simulink model "sinePWM"  (R2024b)
settings: Solver=VariableStepAuto  StartTime=0.0  StopTime=0.5  RelTol=1e-3
libraries: spsMosfetLib x4, spsDCVoltageSourceLib x1, spsSeriesRLCBranchLib x1, spsTriangleGeneratorLib x1, spsVoltageMeasurementLib x1, sps_lib x1
settings Model: Creator=lenovo  LastModifiedBy=lenovo

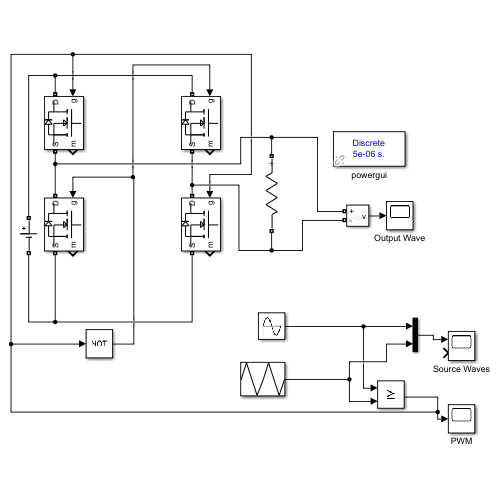
[thumbnail: Simulink's stored preview of the top-level diagram]
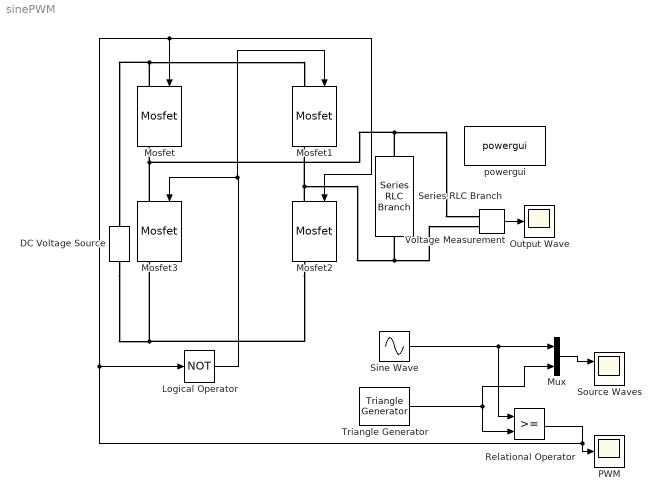
== system sinePWM ==
  DC Voltage Source : spsDCVoltageSourceLib/DC Voltage Source  Amplitude=100  Measurements=None
  Logical Operator : Logic  Operator=NOT  AllPortsSameDT=off  OutDataTypeStr=boolean
  Mosfet{,1..3} (4 alike) : spsMosfetLib/Mosfet  Ron=0.1  Lon=0  Rd=0.01  Vfd=0  IC=0  Rs=1e5  Cs=inf  Measurements=on
  Mux : Mux  Inputs=2
  Output Wave : Scope
  PWM : Scope
  Relational Operator : RelationalOperator  OutDataTypeStr=boolean  RndMeth=Simplest  InputSameDT=off
  Series RLC Branch : spsSeriesRLCBranchLib/Series RLC Branch  LConnTagsString=__new0  RConnTagsString=__new0  BranchType=R  Resistance=1  Inductance=1e-3  SetiL0=off  InitialCurrent=0  Capacitance=1e-6  Setx0=off  InitialVoltage=0  Measurements=None
  Sine Wave : Sin  Frequency=100  SampleTime=0
  Source Waves : Scope  NumInputPorts=2
  Triangle Generator : spsTriangleGeneratorLib/Triangle Generator  Freq=1e1  Phase=90  Ts=0
  Voltage Measurement : spsVoltageMeasurementLib/Voltage Measurement  PhasorSimulation=off  OutputType=Complex  PSBequivalent=0
  powergui : sps_lib/powergui  Priority=1  SimulationMode=Discrete  SampleTime=5e-6  frequency=60  Iterations=50  frequencyindice=0  Pbase=100e6  ErrMax=1e-4  UnitsV=kV  UnitsW=MW  buscounter=0  FunctionMessages=off  echomessages=off  EnableUseOfTLC=off  CurrentSourceSwitches=off  DisableSnubberDevices=off  DisableRonSwitches=off  DisableVfSwitches=off  DisplayEquations=off  AutomaticDiscreteSolvers=off  SolverType=Tustin/Backward Euler (TBE)  Interpol=off  ExternalGateDelay=off  methode=off  Ts=100  x0status=blocks  SPID=on  SwTol=0  HookPort=off  NonlinearTolerance=1e-4  nMaxIteration=100  ContinueOnMaxIteration=off  RestoreLinks=warning  ResistiveCurrentMeasurement=off  Frange=[0:2:500]  Ylog=off  Xlog=on  ShowGrid=off  save=off  variable=ZData  structure=0  ZoomFFT=off  StartTime=0.0  cycles=1  DisplayStyle=1  fundamental=60  FreqAxis=off  MaxFrequency=1000  frequencyindicesteady=1  RmsSteady=1  display=off
  wires:
  Sine Wave/1 -> Relational Operator/1, Mux/1
  Triangle Generator/1 -> Mux/2, Relational Operator/2
  Mux/1 -> Source Waves/1
  Relational Operator/1 -> PWM/1, Mosfet/1, Mosfet2/1, Logical Operator/1
  Logical Operator/1 -> Mosfet3/1, Mosfet1/1
  Voltage Measurement/1 -> Output Wave/1
  connections:
  DC Voltage Source/LConn1 -- Mosfet2/RConn1 -- Mosfet3/RConn1
  Mosfet3/LConn1 -- Voltage Measurement/LConn1 -- Series RLC Branch/LConn1 -- Mosfet/RConn1
  Mosfet2/LConn1 -- Voltage Measurement/LConn2 -- Series RLC Branch/RConn1 -- Mosfet1/RConn1
  Mosfet/LConn1 -- Mosfet1/LConn1 -- DC Voltage Source/RConn1
